simulink model "RonTrap_fig12"  (R2022b)
settings: Solver=ode15s  StartTime=-14  StopTime=39  MaxStep=0.025  RelTol=1e-7  AbsTol=1e-8
settings Model: Creator=Greatlovers  LastModifiedBy=Greatlovers

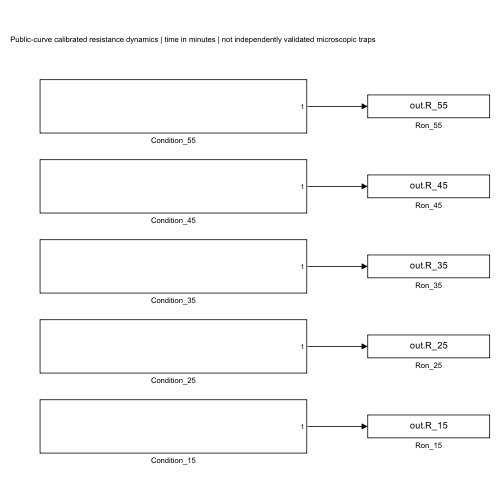
[thumbnail: Simulink's stored preview of the top-level diagram]
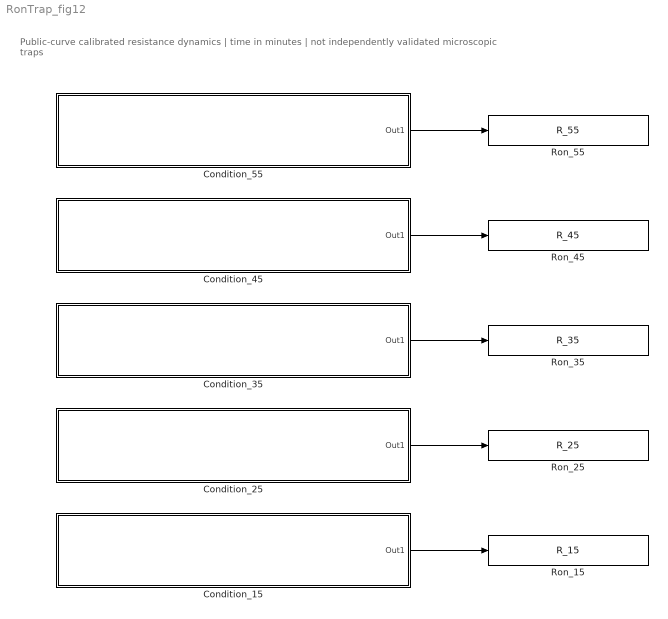
== system RonTrap_fig12 ==
  note: Public-curve calibrated resistance dynamics | time in minutes | not independently validated microscopic traps
  Condition_15 : Subsystem
  Condition_25 : Subsystem
  Condition_35 : Subsystem
  Condition_45 : Subsystem
  Condition_55 : Subsystem
  Ron_15 : ToWorkspace  VariableName=R_15  SaveFormat=Timeseries  SampleTime=-1
  Ron_25 : ToWorkspace  VariableName=R_25  SaveFormat=Timeseries  SampleTime=-1
  Ron_35 : ToWorkspace  VariableName=R_35  SaveFormat=Timeseries  SampleTime=-1
  Ron_45 : ToWorkspace  VariableName=R_45  SaveFormat=Timeseries  SampleTime=-1
  Ron_55 : ToWorkspace  VariableName=R_55  SaveFormat=Timeseries  SampleTime=-1
  wires:
  Condition_55/1(Out1) -> Ron_55/1
  Condition_45/1(Out1) -> Ron_45/1
  Condition_35/1(Out1) -> Ron_35/1
  Condition_25/1(Out1) -> Ron_25/1
  Condition_15/1(Out1) -> Ron_15/1

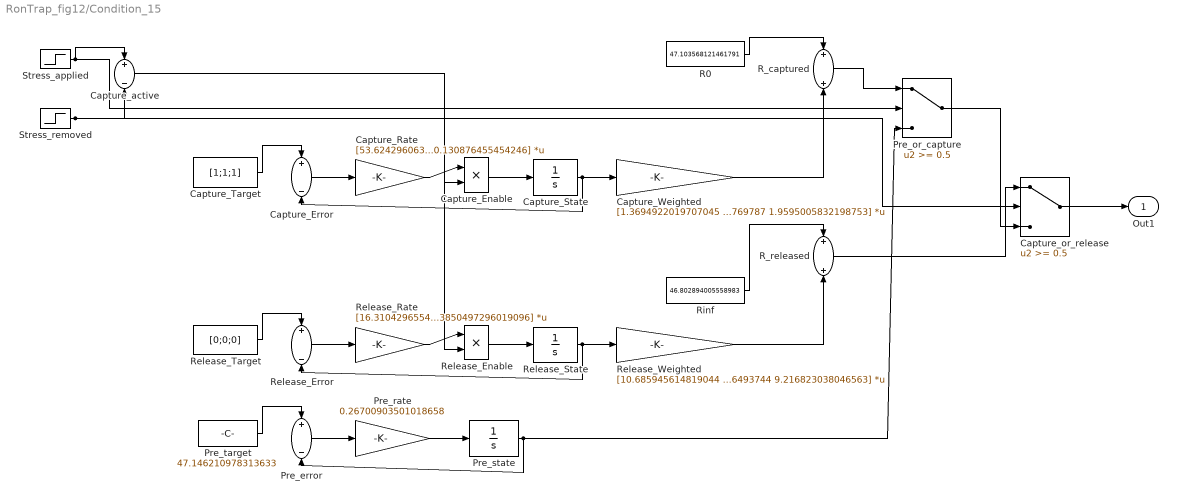
== system RonTrap_fig12/Condition_15 ==
  Capture_Enable : Product  Inputs=**
  Capture_Error : Sum  Inputs=+-
  Capture_Rate : Gain  Gain=[53.624296063815308 0 0;0 2.61837231238363 0;0 0 0.130876455454246]  Multiplication=Matrix(K*u)
  Capture_State : Integrator  InitialCondition=[0;0;0]
  Capture_Target : Constant  Value=[1;1;1]
  Capture_Weighted : Gain  Gain=[1.3694922019707045 21.755580655769787 1.9595005832198753]  Multiplication=Matrix(K*u)
  Capture_active : Sum  Inputs=+-
  Capture_or_release : Switch  Threshold=0.5  SaturateOnIntegerOverflow=off  InputSameDT=off
  Pre_error : Sum  Inputs=+-
  Pre_or_capture : Switch  Threshold=0.5  SaturateOnIntegerOverflow=off  InputSameDT=off
  Pre_rate : Gain  Gain=0.26700903501018658
  Pre_state : Integrator  InitialCondition=45.385999715953972
  Pre_target : Constant  Value=47.146210978313633
  R0 : Constant  Value=47.103568121461791
  R_captured : Sum
  R_released : Sum
  Release_Enable : Product  Inputs=**
  Release_Error : Sum  Inputs=+-
  Release_Rate : Gain  Gain=[16.310429655465388 0 0;0 2.8905116925337113 0;0 0 0.23850497296019096]  Multiplication=Matrix(K*u)
  Release_State : Integrator  InitialCondition=[1;1;1]
  Release_Target : Constant  Value=[0;0;0]
  Release_Weighted : Gain  Gain=[10.685945614819044 5.1654217876493744 9.216823038046563]  Multiplication=Matrix(K*u)
  Rinf : Constant  Value=46.802894005558983
  Stress_applied : Step  Time=-0.066653740142503234  SampleTime=0
  Stress_removed : Step  Time=13.850005093208182  SampleTime=0
  Out1 : Outport
  wires:
  Stress_applied/1 -> Capture_active/1, Pre_or_capture/2
  Stress_removed/1 -> Capture_active/2, Release_Enable/2, Capture_or_release/2
  Capture_Target/1 -> Capture_Error/1
  Capture_State/1 -> Capture_Error/2, Capture_Weighted/1
  Capture_Error/1 -> Capture_Rate/1
  Capture_Rate/1 -> Capture_Enable/1
  Capture_Enable/1 -> Capture_State/1
  Release_Target/1 -> Release_Error/1
  Release_State/1 -> Release_Error/2, Release_Weighted/1
  Release_Error/1 -> Release_Rate/1
  Release_Rate/1 -> Release_Enable/1
  Release_Enable/1 -> Release_State/1
  Capture_active/1 -> Capture_Enable/2
  R0/1 -> R_captured/1
  Capture_Weighted/1 -> R_captured/2
  Rinf/1 -> R_released/1
  Release_Weighted/1 -> R_released/2
  Pre_target/1 -> Pre_error/1
  Pre_state/1 -> Pre_error/2, Pre_or_capture/3
  Pre_error/1 -> Pre_rate/1
  Pre_rate/1 -> Pre_state/1
  R_captured/1 -> Pre_or_capture/1
  R_released/1 -> Capture_or_release/1
  Pre_or_capture/1 -> Capture_or_release/3
  Capture_or_release/1 -> Out1/1

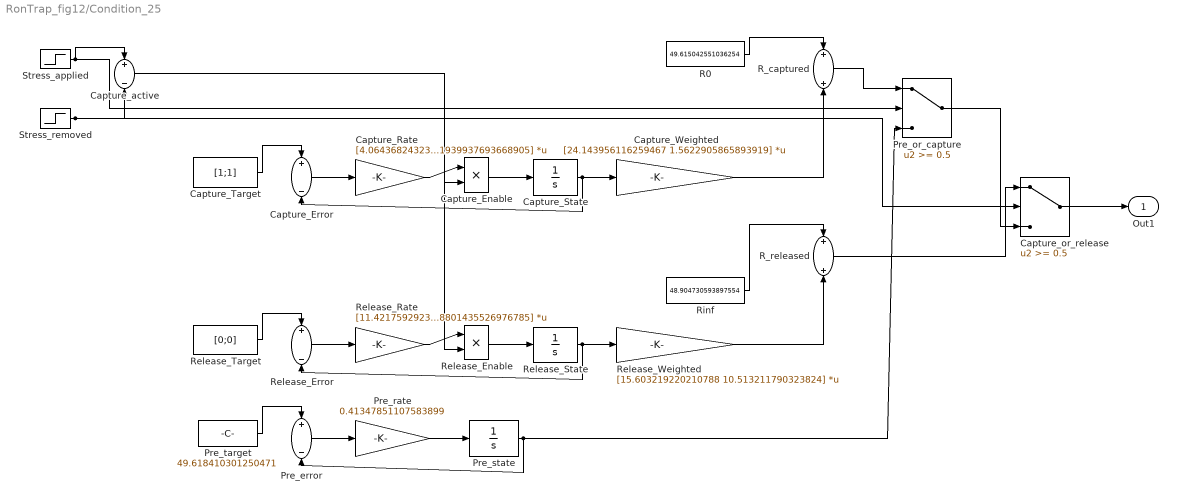
== system RonTrap_fig12/Condition_25 ==
  Capture_Enable : Product  Inputs=**
  Capture_Error : Sum  Inputs=+-
  Capture_Rate : Gain  Gain=[4.0643682432347479 0;0 0.11939937693668905]  Multiplication=Matrix(K*u)
  Capture_State : Integrator  InitialCondition=[0;0]
  Capture_Target : Constant  Value=[1;1]
  Capture_Weighted : Gain  Gain=[24.143956116259467 1.5622905865893919]  Multiplication=Matrix(K*u)
  Capture_active : Sum  Inputs=+-
  Capture_or_release : Switch  Threshold=0.5  SaturateOnIntegerOverflow=off  InputSameDT=off
  Pre_error : Sum  Inputs=+-
  Pre_or_capture : Switch  Threshold=0.5  SaturateOnIntegerOverflow=off  InputSameDT=off
  Pre_rate : Gain  Gain=0.41347851107583899
  Pre_state : Integrator  InitialCondition=48.548442114467854
  Pre_target : Constant  Value=49.618410301250471
  R0 : Constant  Value=49.615042551036254
  R_captured : Sum
  R_released : Sum
  Release_Enable : Product  Inputs=**
  Release_Error : Sum  Inputs=+-
  Release_Rate : Gain  Gain=[11.421759292332117 0;0 0.38801435526976785]  Multiplication=Matrix(K*u)
  Release_State : Integrator  InitialCondition=[1;1]
  Release_Target : Constant  Value=[0;0]
  Release_Weighted : Gain  Gain=[15.603219220210788 10.513211790323824]  Multiplication=Matrix(K*u)
  Rinf : Constant  Value=48.904730593897554
  Stress_applied : Step  Time=-0.066653740142503234  SampleTime=0
  Stress_removed : Step  Time=13.750005174136403  SampleTime=0
  Out1 : Outport
  wires:
  Stress_applied/1 -> Capture_active/1, Pre_or_capture/2
  Stress_removed/1 -> Capture_active/2, Release_Enable/2, Capture_or_release/2
  Capture_Target/1 -> Capture_Error/1
  Capture_State/1 -> Capture_Error/2, Capture_Weighted/1
  Capture_Error/1 -> Capture_Rate/1
  Capture_Rate/1 -> Capture_Enable/1
  Capture_Enable/1 -> Capture_State/1
  Release_Target/1 -> Release_Error/1
  Release_State/1 -> Release_Error/2, Release_Weighted/1
  Release_Error/1 -> Release_Rate/1
  Release_Rate/1 -> Release_Enable/1
  Release_Enable/1 -> Release_State/1
  Capture_active/1 -> Capture_Enable/2
  R0/1 -> R_captured/1
  Capture_Weighted/1 -> R_captured/2
  Rinf/1 -> R_released/1
  Release_Weighted/1 -> R_released/2
  Pre_target/1 -> Pre_error/1
  Pre_state/1 -> Pre_error/2, Pre_or_capture/3
  Pre_error/1 -> Pre_rate/1
  Pre_rate/1 -> Pre_state/1
  R_captured/1 -> Pre_or_capture/1
  R_released/1 -> Capture_or_release/1
  Pre_or_capture/1 -> Capture_or_release/3
  Capture_or_release/1 -> Out1/1

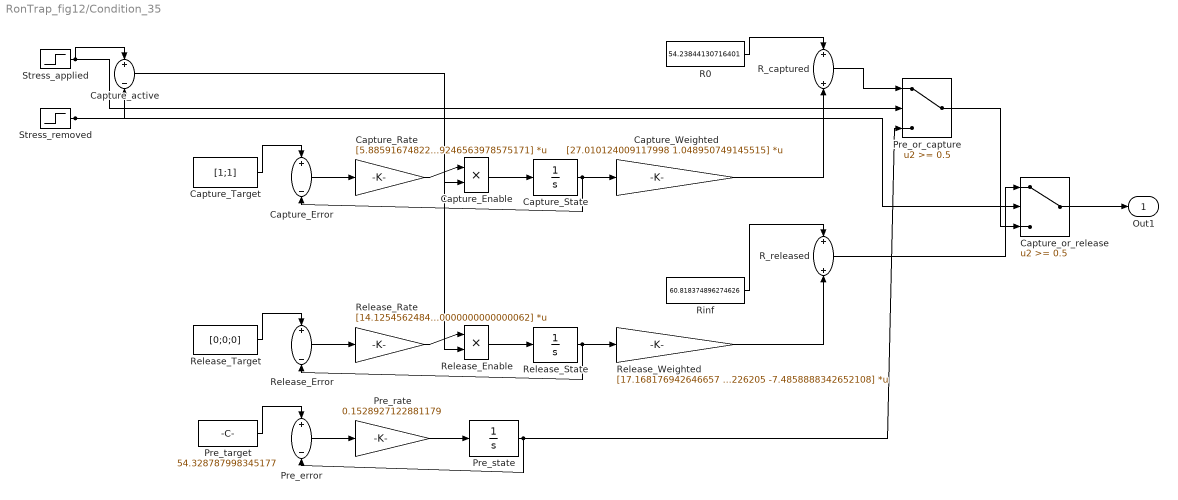
== system RonTrap_fig12/Condition_35 ==
  Capture_Enable : Product  Inputs=**
  Capture_Error : Sum  Inputs=+-
  Capture_Rate : Gain  Gain=[5.8859167482282642 0;0 0.19246563978575171]  Multiplication=Matrix(K*u)
  Capture_State : Integrator  InitialCondition=[0;0]
  Capture_Target : Constant  Value=[1;1]
  Capture_Weighted : Gain  Gain=[27.010124009117998 1.048950749145515]  Multiplication=Matrix(K*u)
  Capture_active : Sum  Inputs=+-
  Capture_or_release : Switch  Threshold=0.5  SaturateOnIntegerOverflow=off  InputSameDT=off
  Pre_error : Sum  Inputs=+-
  Pre_or_capture : Switch  Threshold=0.5  SaturateOnIntegerOverflow=off  InputSameDT=off
  Pre_rate : Gain  Gain=0.1528927122881179
  Pre_state : Integrator  InitialCondition=53.568299114223592
  Pre_target : Constant  Value=54.328787998345177
  R0 : Constant  Value=54.23844130716401
  R_captured : Sum
  R_released : Sum
  Release_Enable : Product  Inputs=**
  Release_Error : Sum  Inputs=+-
  Release_Rate : Gain  Gain=[14.125456248442273 0 0;0 0.57381614874169673 0;0 0 0.0050000000000000062]  Multiplication=Matrix(K*u)
  Release_State : Integrator  InitialCondition=[1;1;1]
  Release_Target : Constant  Value=[0;0;0]
  Release_Weighted : Gain  Gain=[17.168176942646657 11.72619724226205 -7.4858888342652108]  Multiplication=Matrix(K*u)
  Rinf : Constant  Value=60.818374896274626
  Stress_applied : Step  Time=-0.066653740142503234  SampleTime=0
  Stress_removed : Step  Time=13.950005012279961  SampleTime=0
  Out1 : Outport
  wires:
  Stress_applied/1 -> Capture_active/1, Pre_or_capture/2
  Stress_removed/1 -> Capture_active/2, Release_Enable/2, Capture_or_release/2
  Capture_Target/1 -> Capture_Error/1
  Capture_State/1 -> Capture_Error/2, Capture_Weighted/1
  Capture_Error/1 -> Capture_Rate/1
  Capture_Rate/1 -> Capture_Enable/1
  Capture_Enable/1 -> Capture_State/1
  Release_Target/1 -> Release_Error/1
  Release_State/1 -> Release_Error/2, Release_Weighted/1
  Release_Error/1 -> Release_Rate/1
  Release_Rate/1 -> Release_Enable/1
  Release_Enable/1 -> Release_State/1
  Capture_active/1 -> Capture_Enable/2
  R0/1 -> R_captured/1
  Capture_Weighted/1 -> R_captured/2
  Rinf/1 -> R_released/1
  Release_Weighted/1 -> R_released/2
  Pre_target/1 -> Pre_error/1
  Pre_state/1 -> Pre_error/2, Pre_or_capture/3
  Pre_error/1 -> Pre_rate/1
  Pre_rate/1 -> Pre_state/1
  R_captured/1 -> Pre_or_capture/1
  R_released/1 -> Capture_or_release/1
  Pre_or_capture/1 -> Capture_or_release/3
  Capture_or_release/1 -> Out1/1

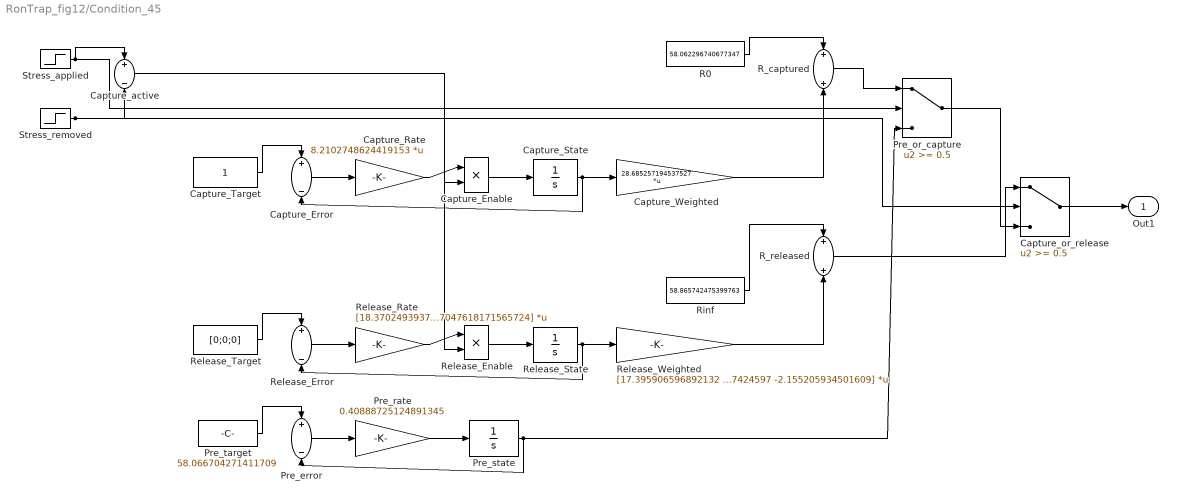
== system RonTrap_fig12/Condition_45 ==
  Capture_Enable : Product  Inputs=**
  Capture_Error : Sum  Inputs=+-
  Capture_Rate : Gain  Gain=8.2102748624419153  Multiplication=Matrix(K*u)
  Capture_State : Integrator
  Capture_Target : Constant
  Capture_Weighted : Gain  Gain=28.685257194537527  Multiplication=Matrix(K*u)
  Capture_active : Sum  Inputs=+-
  Capture_or_release : Switch  Threshold=0.5  SaturateOnIntegerOverflow=off  InputSameDT=off
  Pre_error : Sum  Inputs=+-
  Pre_or_capture : Switch  Threshold=0.5  SaturateOnIntegerOverflow=off  InputSameDT=off
  Pre_rate : Gain  Gain=0.40888725124891345
  Pre_state : Integrator  InitialCondition=56.762083704699144
  Pre_target : Constant  Value=58.066704271411709
  R0 : Constant  Value=58.062296740677347
  R_captured : Sum
  R_released : Sum
  Release_Enable : Product  Inputs=**
  Release_Error : Sum  Inputs=+-
  Release_Rate : Gain  Gain=[18.370249393765068 0 0;0 0.88458674113662761 0;0 0 0.037047618171565724]  Multiplication=Matrix(K*u)
  Release_State : Integrator  InitialCondition=[1;1;1]
  Release_Target : Constant  Value=[0;0;0]
  Release_Weighted : Gain  Gain=[17.395906596892132 12.641110797424597 -2.155205934501609]  Multiplication=Matrix(K*u)
  Rinf : Constant  Value=58.865742475399763
  Stress_applied : Step  Time=-0.083320284111094337  SampleTime=0
  Stress_removed : Step  Time=13.933338337259313  SampleTime=0
  Out1 : Outport
  wires:
  Stress_applied/1 -> Capture_active/1, Pre_or_capture/2
  Stress_removed/1 -> Capture_active/2, Release_Enable/2, Capture_or_release/2
  Capture_Target/1 -> Capture_Error/1
  Capture_State/1 -> Capture_Error/2, Capture_Weighted/1
  Capture_Error/1 -> Capture_Rate/1
  Capture_Rate/1 -> Capture_Enable/1
  Capture_Enable/1 -> Capture_State/1
  Release_Target/1 -> Release_Error/1
  Release_State/1 -> Release_Error/2, Release_Weighted/1
  Release_Error/1 -> Release_Rate/1
  Release_Rate/1 -> Release_Enable/1
  Release_Enable/1 -> Release_State/1
  Capture_active/1 -> Capture_Enable/2
  R0/1 -> R_captured/1
  Capture_Weighted/1 -> R_captured/2
  Rinf/1 -> R_released/1
  Release_Weighted/1 -> R_released/2
  Pre_target/1 -> Pre_error/1
  Pre_state/1 -> Pre_error/2, Pre_or_capture/3
  Pre_error/1 -> Pre_rate/1
  Pre_rate/1 -> Pre_state/1
  R_captured/1 -> Pre_or_capture/1
  R_released/1 -> Capture_or_release/1
  Pre_or_capture/1 -> Capture_or_release/3
  Capture_or_release/1 -> Out1/1

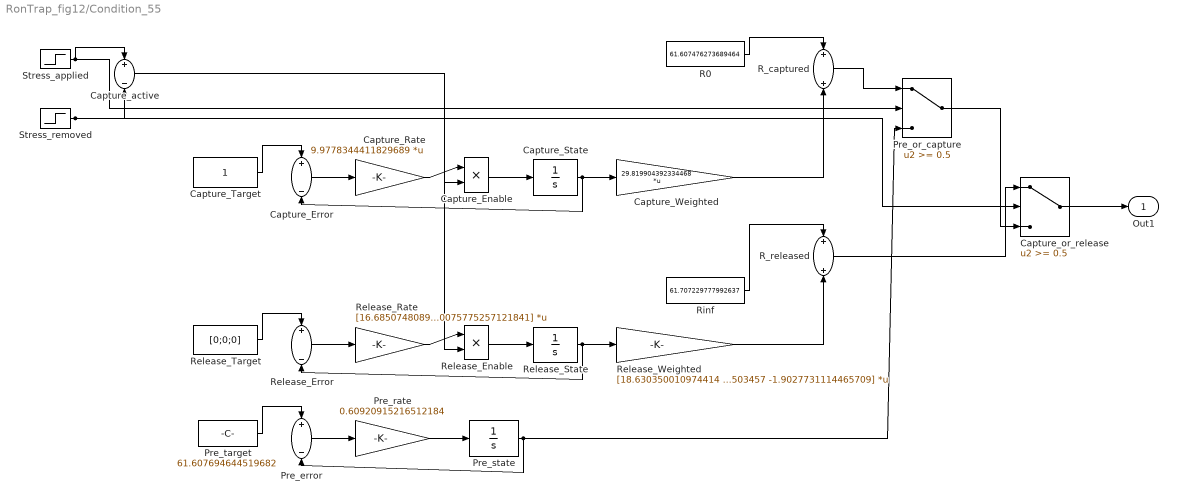
== system RonTrap_fig12/Condition_55 ==
  Capture_Enable : Product  Inputs=**
  Capture_Error : Sum  Inputs=+-
  Capture_Rate : Gain  Gain=9.9778344411829689  Multiplication=Matrix(K*u)
  Capture_State : Integrator
  Capture_Target : Constant
  Capture_Weighted : Gain  Gain=29.819904392334468  Multiplication=Matrix(K*u)
  Capture_active : Sum  Inputs=+-
  Capture_or_release : Switch  Threshold=0.5  SaturateOnIntegerOverflow=off  InputSameDT=off
  Pre_error : Sum  Inputs=+-
  Pre_or_capture : Switch  Threshold=0.5  SaturateOnIntegerOverflow=off  InputSameDT=off
  Pre_rate : Gain  Gain=0.60920915216512184
  Pre_state : Integrator  InitialCondition=60.557628910149944
  Pre_target : Constant  Value=61.607694644519682
  R0 : Constant  Value=61.607476273689464
  R_captured : Sum
  R_released : Sum
  Release_Enable : Product  Inputs=**
  Release_Error : Sum  Inputs=+-
  Release_Rate : Gain  Gain=[16.685074808912542 0 0;0 1.2104780968295301 0;0 0 0.10075775257121841]  Multiplication=Matrix(K*u)
  Release_State : Integrator  InitialCondition=[1;1;1]
  Release_Target : Constant  Value=[0;0;0]
  Release_Weighted : Gain  Gain=[18.630350010974414 12.992573988503457 -1.9027731114465709]  Multiplication=Matrix(K*u)
  Rinf : Constant  Value=61.707229777992637
  Stress_applied : Step  Time=-0.083320284111094337  SampleTime=0
  Stress_removed : Step  Time=13.933338337259313  SampleTime=0
  Out1 : Outport
  wires:
  Stress_applied/1 -> Capture_active/1, Pre_or_capture/2
  Stress_removed/1 -> Capture_active/2, Release_Enable/2, Capture_or_release/2
  Capture_Target/1 -> Capture_Error/1
  Capture_State/1 -> Capture_Error/2, Capture_Weighted/1
  Capture_Error/1 -> Capture_Rate/1
  Capture_Rate/1 -> Capture_Enable/1
  Capture_Enable/1 -> Capture_State/1
  Release_Target/1 -> Release_Error/1
  Release_State/1 -> Release_Error/2, Release_Weighted/1
  Release_Error/1 -> Release_Rate/1
  Release_Rate/1 -> Release_Enable/1
  Release_Enable/1 -> Release_State/1
  Capture_active/1 -> Capture_Enable/2
  R0/1 -> R_captured/1
  Capture_Weighted/1 -> R_captured/2
  Rinf/1 -> R_released/1
  Release_Weighted/1 -> R_released/2
  Pre_target/1 -> Pre_error/1
  Pre_state/1 -> Pre_error/2, Pre_or_capture/3
  Pre_error/1 -> Pre_rate/1
  Pre_rate/1 -> Pre_state/1
  R_captured/1 -> Pre_or_capture/1
  R_released/1 -> Capture_or_release/1
  Pre_or_capture/1 -> Capture_or_release/3
  Capture_or_release/1 -> Out1/1
